simulink model "RoboCup_ARM"  (R2026b)
settings: Solver=FixedStepAuto  StopTime=Inf  FixedStep=0.01
StartFcn:
  | clear attachToRobot
  | clear attachToTool
undefined symbols (not defined in the file or in its folder): gray, q_grip1, Sim3dSensor
libraries: sim3dlib x5, robotsim3dlib x1, robotcorelib x1, robotmaniplib x1, sim3dcameralib x1
settings Model: Creator=Abhishek  LastModifiedBy=liarc_3
settings RTWCC: GPUComputeCapability=5.0

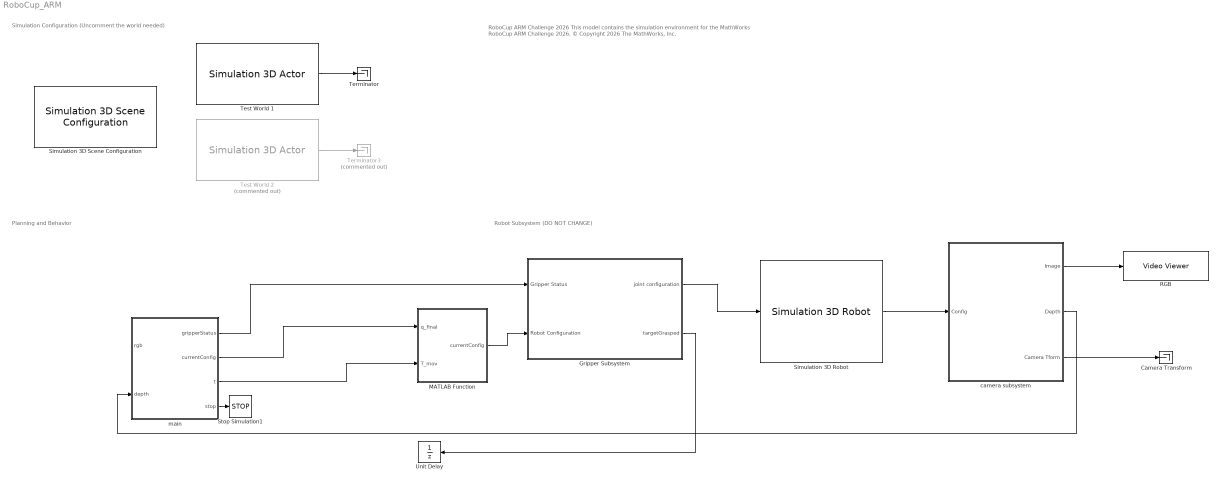
== system RoboCup_ARM ==
  note: Robot Subsystem (DO NOT CHANGE)
  note: Planning and Behavior
  note: Simulation Configuration (Uncomment the world needed)
  note: RoboCup ARM Challenge 2026
      | This model contains the simulation environment for the MathWorks RoboCup ARM Challenge 2026.
      |
      | © Copyright 2026 The MathWorks, Inc.
  Camera Transform : Terminator
  Gripper Subsystem : Subsystem
  MATLAB Function : MATLAB Function  TreatAsAtomicUnit=on
  "RGB " : VideoViewer  colormapValue=gray(256)  FigPos=[431 551 418 304]
  Simulation 3D Robot : robotsim3dlib/Simulation 3D Robot  actorInputType=RigidBodyTree Object  RigidBodyTree=rt.robot  ActorName=Robo1  existActorChekBox=on  initialTrans=[0 0 0]  initialRot=[0 0 0]  initialConfig=[-0.2618 -2.1991 1.9722 -1.3963 -1.5882 1.3265 0 0 0 0 0 0]  EndEffector=right_inner_finger_pad  eeOffsetInpChekBox=off  eeTargetTrans=[0 0 0]  eeTargetRot=[0 0 0]  enableRegionGraspChekBox=off  regionGraspInpChekBox=off  eeTargTransDiff=[0.2 0.2 0.2]  eeTargRotDiff=[0 0 0]  enableVisualVisualization=on  enableCollisionVisualization=off  collisionGeomColor=[0 1 0]  collisionGeomTransp=0.1  inpConfEnbVal=on  inpGraspEnbVal=off  inpTransEnbVal=off  outConfEnbVal=on  outGraspEnbVal=off  outTransEnbVal=off  SampleTime=0.01  ActorType=SimulinkVehicle  ID=C  aMode=6  ActorTag=Robo1  Mesh=RigidBodyTree
  Simulation 3D Scene Configuration : sim3dlib/Simulation 3D Scene Configuration  Priority=0  EnableWindow=on  ViewerType=Default Viewer  ProjectFormat=Default Scenes  SceneDesc=Empty scene  ProjectName=C:\Program Files\MATLAB\R2026b\toolbox\shared\sim3d_projects\automotive_project_windows\UE\WindowsNoEditor\VehicleSimulation.exe  ScenePath=/Game/Maps/HwStrght  EnableOpenDRIVE=off  vehTagList={'Custom';'Robo1';'Scene Origin';'Sim3dActor1';'Sim3dActor2';'Sim3dActor3'}  vehTag=Scene Origin  AttachedCameraRelativeTranslation=[0 0 0]  FreeCameraDefaultInitialTranslation=[-6, 0, 2]  AttachedCameraRelativeRotation=[0 0 0]  FreeCameraDefaultInitialRotation=[0, -15, 0]  ViewpointName=Custom  FreeCameraInitialTranslation=[0, 0, 0]  FreeCameraInitialRotation=[0, 0, 0]  OpVisEn=off  Ts=0.01  EnableRemoteAccess=off  SimulationMode=CoSimulation  SimulateUsing=Interpreted execution  EnableAnimationRecording=off  OverrideDefaultRecording=off  AnimationRecordingFileName=sim3dAnimation.mat  AnimationRecordingInterval=[0 inf]  EnableWeather=off  SunAzimuth=90  SunAltitude=40.0  EnableGeospatialSun=off  Latitude=0  Longitude=0  Date=2023-01-01  Time=10:30:00  GeoTimeZone=-5.0  SunDaylightSaving=off  wind=1  clouds=10  EnableVolumetricClouds=off  CloudCoverage=0  CloudAltitude=6  fog=0  rain=0  RaindropsEffect=off  SnowDensity=0  EnableGeospatial=off  TilesetSource=Earth terrain  UseTrueOrigin=off  OriginHeight=200  OriginLatitude=40.744652  OriginLongitude=-73.988864  MapStyle=Aerial  AdditionalAssetIDs=[]  UseAdvancedSunSky=off  SolarTime=11  TimeZone=-5  Day=21  Month=9  Year=2022  UseDaylightSavingTime=on  DSTStartDay=10  DSTStartMonth=3  DSTEndDay=3  DSTEndMonth=11  DSTSwitchHour=2  sensorTag=MainCamera1  sensorId=1  sensorName=MainCamera1  mountLoc=Origin  offsetFlag=off  tmountOffset=[0, 0, 0]  rmountOffset=[0, 0, 0]  HorizontalResolution=1280  VerticalResolution=720  HorizontalFOV=60  mountPoint=[0 0 0]  mountOrientation=[0 0 0]  aMode=5  ID=1  GeoTrigger=Inactive  ViewNameList={'Custom'}  ViewTranslationList={'[0 0 0]'}  ViewRotationList={'[0 0 0]'}
      settings: LibrarySourceBlock=sl3dlib/Simulation 3D/Environment/Simulation 3D Scene Configuration
  Stop Simulation1 : Stop
  Terminator : Terminator
  Terminator3 : Terminator  Commented=on
  Test World 1 : sim3dlib/Simulation 3D Actor  Priority=1  ActorName=Sim3dActor1  ParentName=Scene Origin  Operation=Create at setup  InitScriptText=|  SampleTime=-1  Translation=[0 0 0]  Rotation=[0 0 0]  Scale=[1 1 1]  aMode=5  ActorTag=Sim3dActor1  ActorType=Sim3dActor  ID=1
      | % Reserved keywords:
      | % - Actor : handle to this actor object
      | % - World : handle to the world object
      | 
      | % Examples:
      | 
      | % Create a primitive geometry (optional)
      | % createShape(Actor, 'box', [1 1 1]);
      | 
      | % Initialize values (optional)
      | % Actor.Physics = true;
      | % Actor.Color = [1 0 0];
      | Actor.load('example_world.mat')
  Test World 2 : sim3dlib/Simulation 3D Actor  Priority=1  Commented=on  ActorName=Sim3dActor3  ParentName=Scene Origin  Operation=Create at setup  InitScriptText=|  SampleTime=-1  Translation=[0 0 0]  Rotation=[0 0 0]  Scale=[1 1 1]  aMode=5  ActorTag=Sim3dActor3  ActorType=Sim3dActor  ID=3
      | % Reserved keywords:
      | % - Actor : handle to this actor object
      | % - World : handle to the world object
      | 
      | % Examples:
      | 
      | % Create a primitive geometry (optional)
      | % createShape(Actor, 'box', [1 1 1]);
      | 
      | % Initialize values (optional)
      | % Actor.Physics = true;
      | % Actor.Color = [1 0 0];
      | Actor.load('example_world2.mat')
  Unit Delay : UnitDelay  SampleTime=-1
  camera subsystem : Subsystem
  main : Stateflow chart  TreatAsAtomicUnit=on
      settings: PortSchema="{\"entries\":[{\"content\":{\"sides\":[{\"content\":{\"connectorIds\":[\"In1\",\"In2\"]},\"type\":\"ConnectorPlacement.EquallySpacedRectSide\",\"uuid\":\"4d732dd7-062d-4689-9f8b-43f99dfb8420\"},{\"content\":{\"connectorIds\":[\"Out1\",\"Out3\",\"Out4\",\"Out2\"],\"side\":\"RIGHT\"},\"type\":\"ConnectorPlacement.EquallySpacedRectSide\",\"uuid\":\"91537844-c947-4718-a544-564235b069fc\"},{\"content\":{\"side\":\"TOP\"},\"type\":\"ConnectorPlacement.EquallySpacedRectSide\",\"uuid\":\"70235710-0307-4145-b826-1629146d59e2\"}]},\"type\":\"ConnectorPlacement.EquallySpacedConnector\",\"uuid\":\"5e015d6f-0741-40bb-ac97-ef390eff1351\"}],\"packageUris\":[\"http://schema.mathworks.com/mf0/Connector/R2020b\"],\"version\":\"1.0\"}"
  wires:
  Gripper Subsystem/1(joint configuration) -> Simulation 3D Robot/1
  Simulation 3D Robot/1 -> camera subsystem/1(Config)
  Gripper Subsystem/2(targetGrasped) -> Unit Delay/1
  Test World 1/1 -> Terminator/1
  camera subsystem/1(Image) -> "RGB "/1
  camera subsystem/2(Depth) -> main/2(depth)
  camera subsystem/3(Camera Tform) -> Camera Transform/1
  Test World 2/1 -> Terminator3/1
  main/2(stop) -> Stop Simulation1/1
  main/1(gripperStatus) -> Gripper Subsystem/1(Gripper Status)
  main/4(t) -> MATLAB Function/2(T_mov)
  main/3(currentConfig) -> MATLAB Function/1(q_final)
  MATLAB Function/1(currentConfig) -> Gripper Subsystem/2(Robot Configuration)

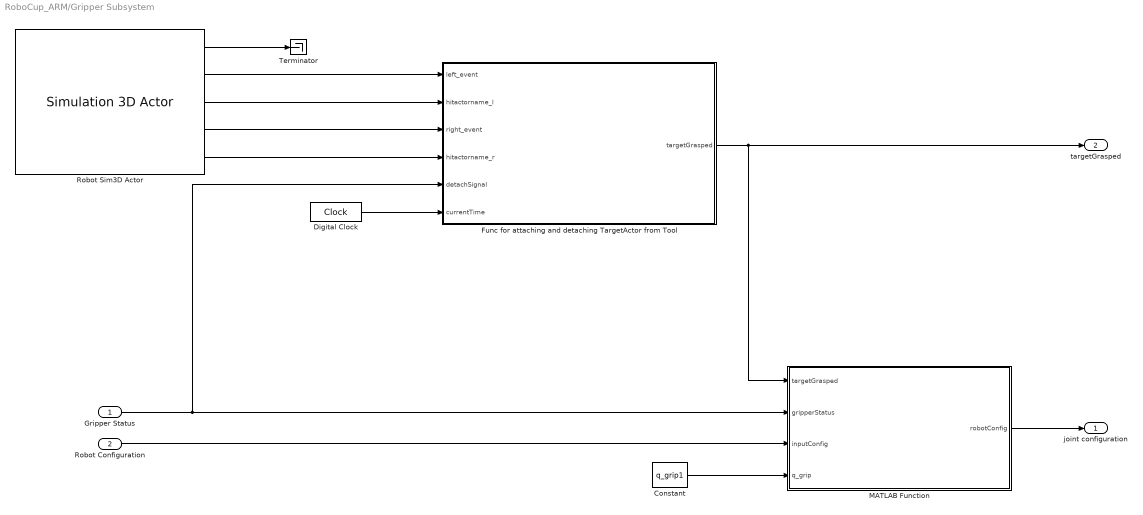
== system RoboCup_ARM/Gripper Subsystem ==
  Gripper Status : Inport
  Robot Configuration : Inport  Port=2
  Constant : Constant  Value=q_grip1
  Digital Clock : DigitalClock
  Func for attaching and detaching TargetActor from Tool : MATLAB Function  TreatAsAtomicUnit=on
  MATLAB Function : MATLAB Function  TreatAsAtomicUnit=on
  Robot Sim3D Actor : sim3dlib/Simulation 3D Actor  Priority=1  ActorName=Sim3dActor2  ParentName=Scene Origin  Operation=Create at setup  InitScriptText=|  SampleTime=-1  Translation=[-0.5 0 1.35]  Rotation=[0 0 0]  Scale=[1 1 1]  EventsText=|  aMode=5  ActorTag=Sim3dActor2  ActorType=Sim3dActor  ID=2
      InitScriptText=|
      | rt = load('ur5e_gripper.mat');
      | robotActor = sim3d.Actor('ActorName', 'Robo1');
      | World.add(robotActor,Actor);
      | 
      | robotActor.load(rt.robot,[1 1 1]);
      | 
      | % finding tool reference 
      | tool1 = World.Actors.left_inner_finger_pad;
      | tool2 = World.Actors.right_inner_finger_pad;
      | tool1.HitEventEnabled = true;
      | tool1.Collisions = true;
      | 
      | tool2.HitEventEnabled = true;
      | tool2.Collisions = true;
      | 
      | %tool1.Physics = true; % somehow this Phsyics dont work
      | % tool1.Color = [10 0 0];
      | tool1.Mobility =  sim3d.utils.MobilityTypes.Movable;
      | 
      | % tool2.Color = [10 0 0];
      | tool2.Mobility =  sim3d.utils.MobilityTypes.Movable;
      | 
      | propagate(World.Actors.('Sim3dActor2'),'Mobility', sim3d.utils.MobilityTypes.Movable);
      | propagate(World.Actors.('Sim3dActor2'),'Shadows',true);
      EventsText=|
      | left_inner_finger_pad.HitEvent          
      | left_inner_finger_pad.HitOtherActorName 
      | right_inner_finger_pad.HitEvent         
      | right_inner_finger_pad.HitOtherActorName
  Terminator : Terminator
  joint configuration : Outport
  targetGrasped : Outport  Port=2
  wires:
  Robot Sim3D Actor/3 -> Func for attaching and detaching TargetActor from Tool/2(hitactorname_l)
  Robot Sim3D Actor/2 -> Func for attaching and detaching TargetActor from Tool/1(left_event)
  Robot Sim3D Actor/4 -> Func for attaching and detaching TargetActor from Tool/3(right_event)
  Robot Sim3D Actor/5 -> Func for attaching and detaching TargetActor from Tool/4(hitactorname_r)
  Digital Clock/1 -> Func for attaching and detaching TargetActor from Tool/6(currentTime)
  Gripper Status/1 -> Func for attaching and detaching TargetActor from Tool/5(detachSignal), MATLAB Function/2(gripperStatus)
  Robot Configuration/1 -> MATLAB Function/3(inputConfig)
  Func for attaching and detaching TargetActor from Tool/1(targetGrasped) -> MATLAB Function/1(targetGrasped), targetGrasped/1
  Constant/1 -> MATLAB Function/4(q_grip)
  MATLAB Function/1(robotConfig) -> joint configuration/1
  Robot Sim3D Actor/1 -> Terminator/1

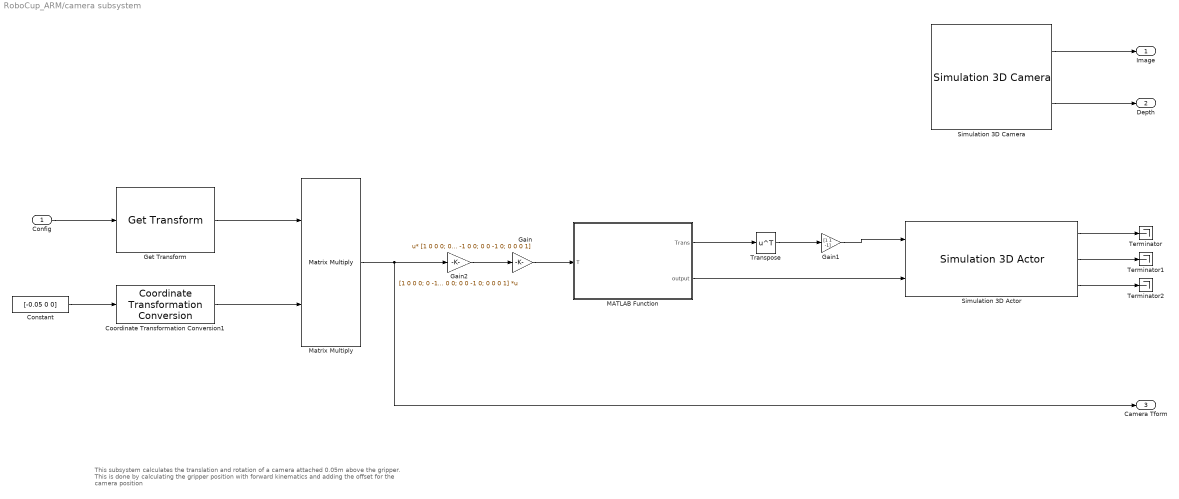
== system RoboCup_ARM/camera subsystem ==
  note: This subsystem calculates the translation and rotation of a camera attached 0.05m above the gripper. This is done by calculating the gripper position with forward kinematics and adding the offset for the camera position
  Config : Inport
  Constant : Constant  Value=[-0.05 0 0]
  Coordinate Transformation Conversion1 : robotcorelib/Coordinate Transformation Conversion  InputRepresentation=Translation Vector  InputEulerSequence=ZYX  ShowTrVecInputPort=on  OutputRepresentation=Homogeneous Transformation  OutputEulerSequence=ZYX  ShowTrVecOutputPort=on  SimulateUsing=Interpreted execution
      settings: LibrarySourceBlock=navlib/Utilities/Coordinate Transformation Conversion
  Gain : Gain  Gain=[1 0 0 0; 0 -1 0 0; 0 0 -1 0; 0 0 0 1]  Multiplication=Matrix(u*K)
  Gain1 : Gain  Gain=[1 1 -1]
  Gain2 : Gain  Gain=[1 0 0 0; 0 -1 0 0; 0 0 -1 0; 0 0 0 1]  Multiplication=Matrix(K*u)
  Get Transform : robotmaniplib/Get Transform  RigidBodyTree=rt.robot  SourceBody=robotiq_arg2f_base_link  TargetBody=base_link  SimulateUsing=Interpreted execution
  MATLAB Function : MATLAB Function  TreatAsAtomicUnit=on
  Matrix Multiply : Product  Multiplication=Matrix(*)
  Simulation 3D Actor : sim3dlib/Simulation 3D Actor  Priority=1  ActorName=cameraPlaceHolder  ParentName=Robo1  Operation=Create at setup  InitScriptText=|  SampleTime=-1  Translation=[0.05 0 0]  Rotation=[0 0 0]  Scale=[1 1 1]  InputsText=cameraPlaceHolder.Translation cameraPlaceHolder.Rotation  OutputsText=cameraPlaceHolder.Translation cameraPlaceHolder.Rotation  aMode=5  ActorTag=cameraPlaceHolder  ActorType=Sim3dActor  ID=C
      | Actor.createShape('box', [0.02 0.04 0.06]);
      | Actor.Mobility=sim3d.utils.MobilityTypes.Movable;
      | Actor.Color=[1 0 0];
      | Actor.Translation=[0.05, 0, 0];
      | Actor.Rotation = [0, 0, 0];
      | Actor.ConstantAttributes=false;
      | Actor.Mass = 1;
      | Actor.Transparency = 0;
      | Actor.Shininess = 0;
  Simulation 3D Camera : sim3dcameralib/Simulation 3D Camera  Priority=1  sensorTag=Sim3dSensor�  sensorId=1  sensorName=Sim3dSensor�  vehTagList={'Robo1';'Scene Origin';'Sim3dActor1';'Sim3dActor2';'Sim3dActor3';'cameraPlaceHolder'}  vehTag=cameraPlaceHolder  CoordinateSystem=ISO8855  mountLoc=Origin  offsetFlag=on  tmountOffset=[0 0 0]  extTmount=off  rmountOffset=[0, -90, 0]  extRmount=off  FocalLength=[1109, 1109]  OpticalCenter=[640, 360]  ImageSize=[720, 1280]  RadialDistortion=[0, 0]  TangentialDistortion=[0, 0]  SensorSkew=0  VisualizeFieldOfView=off  FieldOfViewRange=61  DepthOutportEnabled=on  SemanticOutportEnabled=off  TransformOutportEnabled=off  SampleTime=0.01  mountPoint=[0 0 0]  mountOrientation=[0 -90 0]  aMode=5  ID=1
      settings: LibrarySourceBlock=sl3dlib/Simulation 3D/Sensors/Simulation 3D Camera
  Terminator : Terminator
  Terminator1 : Terminator
  Terminator2 : Terminator
  Transpose : Math  Operator=transpose
  Image : Outport
  Depth : Outport  Port=2
  Camera Tform : Outport  Port=3
  wires:
  MATLAB Function/1(Trans) -> Transpose/1
  Coordinate Transformation Conversion1/1 -> Matrix Multiply/2
  Simulation 3D Actor/2 -> Terminator1/1
  Transpose/1 -> Gain1/1
  Simulation 3D Camera/2 -> Depth/1
  Simulation 3D Actor/1 -> Terminator/1
  Gain/1 -> MATLAB Function/1(T)
  Simulation 3D Actor/3 -> Terminator2/1
  MATLAB Function/2(output) -> Simulation 3D Actor/2
  Matrix Multiply/1 -> Gain2/1, Camera Tform/1
  Gain1/1 -> Simulation 3D Actor/1
  Get Transform/1 -> Matrix Multiply/1
  Simulation 3D Camera/1 -> Image/1
  Gain2/1 -> Gain/1
  Constant/1 -> Coordinate Transformation Conversion1/1
  Config/1 -> Get Transform/1

== matlab function RoboCup_ARM/Gripper Subsystem/MATLAB Function ==
  data: targetGrasped input; robotConfig output; gripperStatus input; inputConfig input; q_grip input
function robotConfig = appendGripper(targetGrasped, gripperStatus, inputConfig, q_grip)

persistent index
if isempty(index)
    index = 1;
end

% Open gripper
if ~gripperStatus
    openConfig = [0 0 0 0 0 0]';
    robotConfig = [inputConfig; openConfig]';
    index = 1;
else
    if index > size(q_grip, 2)
        robotConfig = [inputConfig; q_grip(:, index-1)]';
        index = 1;
    elseif targetGrasped
        robotConfig = [inputConfig; q_grip(:, index)]';
    else
        robotConfig = [inputConfig; q_grip(:, index)]';
        index = index + 1;
    end
end

== matlab function RoboCup_ARM/Gripper Subsystem/Func for attaching and detaching TargetActor from Tool ==
  data: left_event input; targetGrasped output; hitactorname_l input; right_event input; hitactorname_r input; detachSignal input; currentTime input
 function targetGrasped = attachToRobot(left_event, hitactorname_l, right_event, hitactorname_r, detachSignal, currentTime)
    
    persistent l_time r_time grasped;
    if isempty(l_time)
        l_time = 0;
    end

    if isempty(r_time)
        r_time = 1;
    end

    if left_event
        l_time = currentTime;
    end

    if right_event
        r_time = currentTime;
    end
    
    if isempty(grasped)
        grasped = 0;
    end

    targetGrasped = grasped;

    coder.extrinsic('attachToTool');

    if abs(l_time - r_time) < 0.5 || ~detachSignal
        grasped = attachToTool(hitactorname_l, hitactorname_r,detachSignal);
        targetGrasped = grasped;
    end
end

== matlab function RoboCup_ARM/camera subsystem/MATLAB Function ==
  data: T input; Trans output; output output
function [Trans, output] = rotm2fixedZYX(T)
    R = T(1:3,1:3);
    Trans = T(1:3,4);
    if abs(R(3,1)) < 1
        pitch = -asin(R(3,1));
        roll  = atan2(R(3,2)/cos(pitch), R(3,3)/cos(pitch));
        yaw   = atan2(R(2,1)/cos(pitch), R(1,1)/cos(pitch));
    else
        % Gimbal lock
        if R(3,1) <= -1
            pitch = pi/2;
        else
            pitch = -pi/2;
        end
        yaw = 0;
        roll = atan2(-R(1,2), R(1,3));
    end
    output = [roll, pitch, yaw];
end

== stateflow chart RoboCup_ARM/main ==
  state start
    en:
    currentConfig = [0; -pi/2; 0; 0; -pi/2; pi/2];
    gripperStatus = 0;
    stop = false;
    area = 1;
    t = 3;
  state posicao_de_busca
    en:
    pos_busca = [
    0.4 0 0.8; % amarela
    0.1 0.65 0.6; % cinza 1
    -0.05 -0.5 0.6; % cinza 3
    1.35 0 0.8; % vermelho 1
    1.4 -0.9 0.8; %vermelho 2
    0.45 -0.8 0.8; % azul
    0.5 0.65 0.5; % cinza 2
    ];
    pos_garra = pos_busca(area, :);
    [currentConfig, pos_atual,ang_anterior] = pose(pos_garra,currentConfig,0.5,1,0);
  (default) -> start
  start -> posicao_de_busca : after(1,sec)
  data: currentConfig function_output; pos_atual function_output; pos_alvo function_input; chute_inicial function_input; peso_pos function_input; peso_ori function_input; chute_inicial function_output; ang function_input; h function_output; tipo function_input; estado function_input; rgb input; gripperStatus output; stop output; depth input; currentConfig output; pos_busca local; area local; angulo local; estado local; pos_garra local; pos_objeto local; tipo local; h local; t output; pos_atual local; ang_anterior local
  function [currentConfig, pos_atual, chute_inicial] = pose(pos_alvo, chute_inicial, peso_pos, peso_ori, ang):
    | function [currentConfig, pos_atual, chute_inicial] = pose(pos_alvo, chute_inicial, peso_pos, peso_ori, ang)
    | 
    |     % Chute inicial
    |     chute = zeros(1,5);
    |     chute(1) = chute_inicial(1);
    |     chute(2) = chute_inicial(2);
    |     chute(3) = chute_inicial(3);
    |     chute(4) = chute_inicial(4);
    |     chute(5) = chute_inicial(6);
    | 
    |     % Chamando cinemática inversa
    |     coder.extrinsic('cinematica_inversa_generica');
    | 
    |     % Pré-aloca a variável
    |     config_calculada = zeros(1, 6);
    | 
    |     % Chama a sua função para encontrar os ângulos das juntas
    |     [config_calculada, pos_atual] = cinematica_inversa_generica(pos_alvo, chute, peso_pos, peso_ori, ang);
    | 
    |     % Normaliza todos os ângulos para o intervalo [-pi, pi]
    |     config_calculada = mod(config_calculada + pi, 2*pi) - pi;
    | 
    |     % Transforma o resultado em um vetor coluna (6x1)
    |     currentConfig = config_calculada(:);
    | end
  function h = altura(tipo, estado):
    | function h = altura(tipo, estado)
    |     % DEFINIRH Calcula o valor de h com base no tipo e no estado.
    |     % tipo: Inteiro de 1 a 6
    |     % estado: 0 ou 1
    |     
    |     switch tipo
    |         case 1
    |             if estado == 1
    |                 h = 0.18;
    |             else
    |                 h = 0.15;
    |             end
    |             
    |         case 2
    |             if estado == 1
    |                 h = 0.18;
    |             else
    |                 h = 0.15;
    |             end
    |             
    |         case 3
    |             if estado == 1
    |                 h = 0.2;
    |             else
    |                 h = 0.15;
    |             end
    |             
    |         case 4
    |             if estado == 1
    |                 h = +0.08;
    |             else
    |                 h = 0.1;
    |             end
    |             
    |         case {5, 6}
    |             % Para os tipos 5 e 6, h é independente do estado
    |             h = 0.15;
    |             
    |         otherwise
    |             error('Tipo inválido. Insira um valor entre 1 e 6.');
    |     end
    | end

== matlab function RoboCup_ARM/MATLAB Function ==
  data: currentConfig output; q_final input; T_mov input
function currentConfig = generateTraj(q_final, T_mov)
%#codegen

    T_sim = 0.01;
    N = max(round(T_mov / T_sim), 2);

    persistent alpha;
    persistent q_atual;

    % Inicializa na primeira chamada
    if isempty(alpha)
        alpha = 0;
    end

    if isempty(q_atual)
        q_atual = zeros(6, 1);
    end

    % Reset: q_final == q_atual sinaliza nova trajetória
    if norm(q_final - q_atual) < 1e-6
        alpha = 0;
        currentConfig = q_atual;
    else
        % Calcula configuração atual
        currentConfig = q_atual + alpha * (q_final - q_atual);

        % Avança alpha
        if alpha < 1
            alpha = min(alpha + 1/(N - 1), 1);
        end
    end

    % Atualiza q_atual
    q_atual = currentConfig;

end
